simulink model "dq_current_controller"  (R2025b)
settings: Solver=VariableStepAuto  StartTime=0.0  StopTime=10.0  RelTol=1e-3
undefined symbols (not defined in the file): control, motor
settings Model: Creator=semih  LastModifiedBy=semih
settings GRTTargetCC: CombineOutputUpdateFcns=off

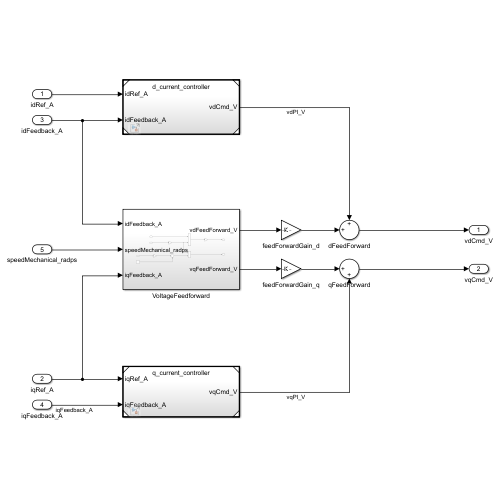
[thumbnail: Simulink's stored preview of the top-level diagram]
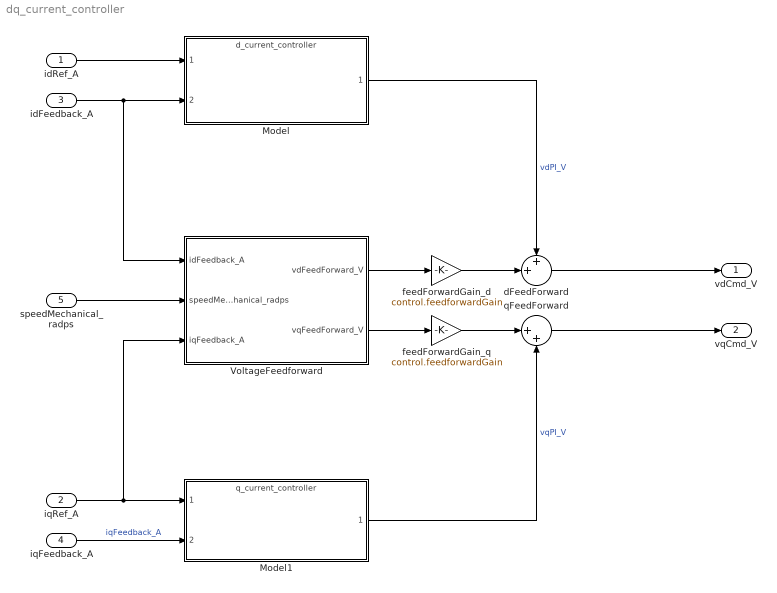
== system dq_current_controller ==
  idRef_A : Inport
  iqRef_A : Inport  Port=2
  idFeedback_A : Inport  Port=3
  iqFeedback_A : Inport  Port=4
  speedMechanical_radps : Inport  Port=5
  Model : ModelReference  ModelNameDialog=d_current_controller  SimulationMode=Normal  ModelReferenceVersion=1.6
  Model1 : ModelReference  ModelNameDialog=q_current_controller  SimulationMode=Normal  ModelReferenceVersion=1.4
  VoltageFeedforward : Subsystem
  dFeedForward : Sum  Inputs=++|
  feedForwardGain_d : Gain  Gain=control.feedforwardGain
  feedForwardGain_q : Gain  Gain=control.feedforwardGain
  qFeedForward : Sum  Inputs=|++
  vdCmd_V : Outport
  vqCmd_V : Outport  Port=2
  wires:
  idRef_A/1 -> Model/1
  idFeedback_A/1 -> Model/2, VoltageFeedforward/1(idFeedback_A)
  iqRef_A/1 -> Model1/1, VoltageFeedforward/3(iqFeedback_A)
  iqFeedback_A/1 -> Model1/2  "iqFeedback_A"
  Model/1 -> dFeedForward/1  "vdPI_V"
  Model1/1 -> qFeedForward/2  "vqPI_V"
  VoltageFeedforward/2(vqFeedForward_V) -> feedForwardGain_q/1
  VoltageFeedforward/1(vdFeedForward_V) -> feedForwardGain_d/1
  qFeedForward/1 -> vqCmd_V/1
  dFeedForward/1 -> vdCmd_V/1
  speedMechanical_radps/1 -> VoltageFeedforward/2(speedMechanical_radps)
  feedForwardGain_q/1 -> qFeedForward/1
  feedForwardGain_d/1 -> dFeedForward/2

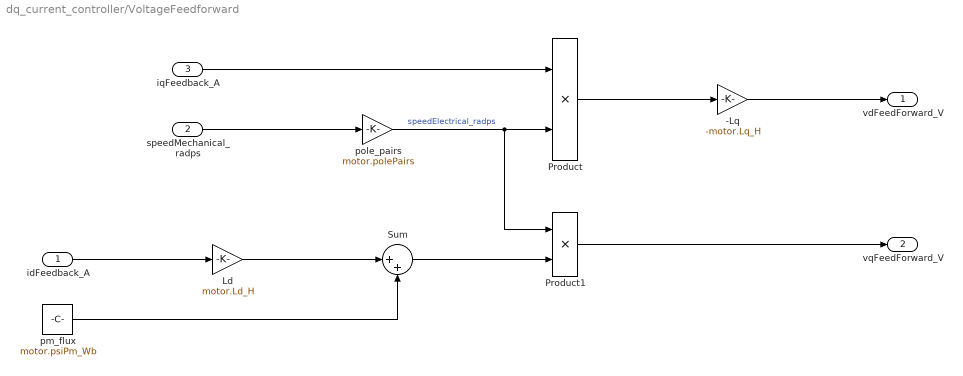
== system dq_current_controller/VoltageFeedforward ==
  idFeedback_A : Inport
  speedMechanical_radps : Inport  Port=2
  iqFeedback_A : Inport  Port=3
  -Lq : Gain  Gain=-motor.Lq_H
  Ld : Gain  Gain=motor.Ld_H
  Product : Product
  Product1 : Product
  Sum : Sum  Inputs=|++
  pm_flux : Constant  Value=motor.psiPm_Wb
  pole_pairs : Gain  Gain=motor.polePairs
  vdFeedForward_V : Outport
  vqFeedForward_V : Outport  Port=2
  wires:
  speedMechanical_radps/1 -> pole_pairs/1
  pole_pairs/1 -> Product1/1, Product/2  "speedElectrical_radps"
  iqFeedback_A/1 -> Product/1
  Product/1 -> -Lq/1
  -Lq/1 -> vdFeedForward_V/1
  idFeedback_A/1 -> Ld/1
  pm_flux/1 -> Sum/2
  Ld/1 -> Sum/1
  Sum/1 -> Product1/2
  Product1/1 -> vqFeedForward_V/1
